simulink model "sm_trackV_belt4_IdlerArm_i2u0r3"  (R2026b)
settings: Solver=ode23t  StopTime=14  AbsTol=1e-3  EnableMultiTasking=on
PostLoadFcn:
  | sm_trackV_measure_loads([bdroot '/Track FL'],'Actuator Torque')
  | sm_trackV_measure_loads([bdroot '/Track FR'],'Actuator Torque')
  | sm_trackV_measure_loads([bdroot '/Track RL'],'Actuator Torque')
  | sm_trackV_measure_loads([bdroot '/Track RR'],'Actuator Torque')
StartFcn:
  | tic
StopFcn:
  | Elapsed_Sim_Time = toc;
  | disp(['Elapsed Sim Time = ' num2str(Elapsed_Sim_Time)]);
undefined symbols (not defined in the file): X, Y, Z
libraries: sm_lib x9, fl_lib x8, nesl_utility x5, sm_trackV_lib_chain_underc_elem x4, simulink x4, sm_trackV_lib_belt_lower_frame_s45i2u0l3 x4, sm_excv_chassis_lib x3, sm_trackV_lib_terrain_contact x3
settings Model: Creator=smiller  LastModifiedBy=smiller
settings SolverCC: AutoScaleAbsTol=off
settings DataIOCC: LimitDataPoints=on  MaxDataPoints=10000  ReturnWorkspaceOutputs=off  SignalLoggingName=logsout_sm_trackV_belt4_IdlerArm_i2u0r3
settings OptimizationCC: LifeSpan=inf  ReuseModelBlockBuffer=off
settings DebuggingCC: AllowSymbolicDim=off  ArithmeticOperatorsInVariantConditions=warning  SFExecutionAtInitializationDiag=none  SFNoUnconditionalDefaultTransitionDiag=warning  SFUnexpectedBacktrackingDiag=warning  SubsystemReferenceDiagnosticForUnitTest=warning
settings SFSimCC: CustomCodeUndefinedFunction=UseInterfaceOnly  SimUseLocalCustomCode=off
settings RTWCC: DLArmComputeVersion=19.05  RTWUseLocalCustomCode=off
settings CodeAppCC: StateflowObjectComments=on
settings GRTTargetCC: TargetLangStandard=C89/C90 (ANSI)
settings ConfigComp: CovExternalEMLEnable=off  CovSFcnEnable=off  CovSaveCumulativeToWorkspaceVar=on  CovSaveSingleToWorkspaceVar=on
settings SimscapeCC: SimscapeLogLimitData=off  SimscapeLogName=simlog_sm_trackV_belt4_IdlerArm_i2u0r3  SimscapeLogSimulationStatistics=on  SimscapeLogType=all  SimscapeUseEnergyAccounting=off
settings DiagnosticsConfigSet: SimMechanicsConflictingReferenceFrames=none  SimMechanicsUnconnectedFramePorts=none
settings ExplorerConfigSet: InternalSimMechanicsExplorerSettings="<ExplorerConfiguration><canonicalview>default</canonicalview><AnimationSetting><BasePlaybackSpeed>1.0</BasePlaybackSpeed><PlaybackSpeedFactor>4.0</PlaybackSpeedFactor></AnimationSetting><TilePanel><TileInfo><Tiles Columns=\"2\" Count=\"3\" Rows=\"2\"><Column Weight=\"0.5\"/><Column Weight=\"0.5\"/><Row Weight=\"0.4992\"/><Row Weight=\"0.5008\"/><Tile Height=\"2\" Width=\"1\" X=\"0\" Y=\"0\"/><Tile Height=\"1\" Width=\"1\" X=\"1\" Y=\"0\"/><Tile Height=\"1\" Width=\"1\" X=\"1\" Y=\"1\"/></Tiles></TileInfo><SceneInfo><SceneViewer><BGColor><R>1</R><G>1</G><B>1</B></BGColor><Camera><DoPerspective>on</DoPerspective><Position><X>8</X><Y>-4.69999999999999929</Y><Z>3.49999999999999956</Z></Position><Center><X>7.32379042217759135</X><Y>-4.02379042217759064</Y><Z>3.20762829527726279</Z></Center><Up><X>0</X><Y>0</Y><Z>1</Z></Up><ViewLimDist>1</ViewLimDist><YLim>0.466307658154998583</YLim><XLim>0.48985854998100864</XLim></Camera></SceneViewer><SceneViewer><BGColor><R>1</R><G>1</G><B>1</B></BGColor><Camera><DoPerspective>on</DoPerspective><Position><X>0</X><Y>-3.99999999999999911</Y><Z>1.09999999999999964</Z></Position><Center><X>2.22044604925031308e-16</X><Y>-2.99999999999999911</Y><Z>1.09999999999999964</Z></Center><Up><X>0</X><Y>0</Y><Z>1</Z></Up><ViewLimDist>1</ViewLimDist><YLim>0.466307658154998583</YLim><XLim>0.996493077701092966</XLim></Camera></SceneViewer><SceneViewer><BGColor><R>1</R><G>1</G><B>1</B></BGColor><Camera><DoPerspective>on</DoPerspective><Position><X>2</X><Y>8.88178419700125232e-16</Y><Z>9</Z></Position><Center><X>2</X><Y>8.88178419700125232e-16</Y><Z>8</Z></Center><Up><X>0</X><Y>1</Y><Z>0</Z></Up><ViewLimDist>1</ViewLimDist><YLim>0.466307658154998583</YLim><XLim>0.993092077435901444</XLim></Camera></SceneViewer></SceneInfo></TilePanel><MechEditorPanel><Cameras><Camera><Id>Camera1</Id><Value><Name>Track_CtrRear_AimFront</Name><NativeCamera><PositionTrackingFeature>Chassis.Camera_Frames.CamF_CtrRear_AimLF.R</PositionTrackingFeature><CenterTrackingFeature>Config.World_Frame.W</CenterTrackingFeature><UpVectorTrackingFeature>Config.World_Frame.W</UpVectorTrackingFeature><CenterTrackingOrigin>off</CenterTrackingOrigin><CenterTrackingDirection>+X</CenterTrackingDirection><UpVectorTrackingDirection>+Z</UpVectorTrackingDirection></NativeCamera></Value></Camera><Camera><Id>Camera2</Id><Value><Name>Track_Left_AimRight</Name><NativeCamera><PositionTrackingFeature>Chassis.Camera_Frames.CamF_Left_AimRight.R</PositionTrackingFeature><CenterTrackingFeature>Chassis.Camera_Frames.CamF_Left_AimRight.R</CenterTrackingFeature><UpVectorTrackingFeature>Config.World_Frame.W</UpVectorTrackingFeature><CenterTrackingOrigin>off</CenterTrackingOrigin><CenterTrackingDirection>+X</CenterTrackingDirection><UpVectorTrackingDirection>+Z</UpVectorTrackingDirection></NativeCamera></Value></Camera><Camera><Id>Camera3</Id><Value><Name>Track_Front_AimLR</Name><NativeCamera><PositionTrackingFeature>Chassis.Camera_Frames.CamF_Front_AimLR.R</PositionTrackingFeature><CenterTrackingFeature>Chassis.Camera_Frames.Transform_Front_AimLR.F</CenterTrackingFeature><UpVectorTrackingFeature>Config.World_Frame.W</UpVectorTrackingFeature><CenterTrackingOrigin>off</CenterTrackingOrigin><CenterTrackingDirection>+X</CenterTrackingDirection><UpVectorTrackingDirection>+Z</UpVectorTrackingDirection></NativeCamera></Value></Camera><Camera><Id>Camera4</Id><Value><Name>Track_Right_AimLeftTL</Name><NativeCamera><PositionTrackingFeature>Chassis.Camera_Frames.CamF_Right_AimLeftTL.R</PositionTrackingFeature><CenterTrackingFeature>Chassis.Camera_Frames.CamF_Right_AimLeftTL.R</CenterTrackingFeature><UpVectorTrackingFeature>Config.World_Frame.W</UpVectorTrackingFeature><CenterTrackingOrigin>off</CenterTrackingOrigin><CenterTrackingDirection>+X</CenterTrackingDirection><UpVectorTrackingDirection>+Z</UpVectorTrackingDirection></NativeCamera></Value></Camera><Camera><Id>Camera5</Id><Value><Name>Track_Right_AimLeftTR</Name><NativeCamera><PositionTrackingFeature>Chassis.Camera_Frames.CamF_Right_AimLeftTR.R</PositionTrackingFeature><CenterTrackingFeature>Chassis.Camera_Frames.CamF_Right_AimLeftTR.R</CenterTrackingFeature><UpVectorTrackingFeature>Config.World_Frame.W</UpVectorTrackingFeature><CenterTrackingOrigin>off</CenterTrackingOrigin><CenterTrackingDirection>+X</CenterTrackingDirection><UpVectorTrackingDirection>+Z</UpVectorTrackingDirection></NativeCamera></Value></Camera><Camera><Id>Camera6</Id><Value><Name>Track_FR_AimFront</Name><NativeCamera><PositionTrackingFeature>Chassis.Camera_Frames.CamF_FR_Aim_Front_R</PositionTrackingFeature><CenterTrackingFeature>Chassis.Camera_Frames.CamF_FR_Aim_Front_R</CenterTrackingFeature><UpVectorTrackingFeature>Config.W</UpVectorTrackingFeature><CenterTrackingOrigin>off</CenterTrackingOrigin><CenterTrackingDirection>+X</CenterTrackingDirection><UpVectorTrackingDirection>+Z</UpVectorTrackingDirection></NativeCamera></Value></Camera><Camera><Id>Camera7</Id><Value><Name>TrackIsoFR</Name><NativeCamera><PositionKeyframeSet><Keyframe><Time>0</Time><Value><X>7.6744465174951229</X><Y>-7.3378434494995588</Y><Z>0.83192924808838675</Z></Value></Keyframe><Keyframe><Time>4.8580359639439301</Time><Value><X>7.6744465174951229</X><Y>-7.3378434494995588</Y><Z>0.83192924808838675</Z></Value></Keyframe><Keyframe><Time>7.0422197385672698</Time><Value><X>8.4041500304882533</X><Y>-6.0478565656515233</Y><Z>1.2378387423585568</Z></Value></Keyframe><Keyframe><Time>12.78196840006439</Time><Value><X>20.29732183415512</X><Y>-9.1045432763174095</Y><Z>1.6217023498793322</Z></Value></Keyframe></PositionKeyframeSet><CenterKeyframeSet><Keyframe><Time>0</Time><Value><X>-3.9707986865367024</X><Y>13.1242688081241</Y><Z>1.8580696339996621</Z></Value></Keyframe><Keyframe><Time>4.8580359639439301</Time><Value><X>4.507312599752261</X><Y>-1.7728039312810333</Y><Z>1.1110065851169071</Z></Value></Keyframe><Keyframe><Time>7.0422197385672698</Time><Value><X>6.9754199629584264</X><Y>-2.3648388994835718</Y><Z>1.2924635728623486</Z></Value></Keyframe><Keyframe><Time>12.78196840006439</Time><Value><X>16.536524754348189</X><Y>-2.4963653739311518</Y><Z>1.9530913158644347</Z></Value></Keyframe></CenterKeyframeSet><UpVectorKeyframeSet><Keyframe><Time>0</Time><Value><X>0.036204453435340365</X><Y>-0.029489201528742272</Y><Z>0.99890921736894867</Z></Value></Keyframe><Keyframe><Time>4.8580359639439301</Time><Value><X>0.036204453435340372</X><Y>-0.029489201528742279</Y><Z>0.99890921736894867</Z></Value></Keyframe><Keyframe><Time>7.0422197385672698</Time><Value><X>0.015774113925201387</X><Y>-0.0087099802030477149</Y><Z>0.99983764360756966</Z></Value></Keyframe><Keyframe><Time>12.78196840006439</Time><Value><X>0.036204453435340372</X><Y>-0.029489201528742286</Y><Z>0.99890921736894867</Z></Value></Keyframe></UpVectorKeyframeSet></NativeCamera></Value></Camera><Camera><Id>Camera8</Id><Value><Name>Track_IsoFR_Big</Name><NativeCamera><PositionTrackingFeature>Chassis.Camera_Frames.CamF_FR_AimCtr_Big.R</PositionTrackingFeature><CenterTrackingFeature>Chassis.Camera_Frames.CamF_FR_AimCtr_Big.R</CenterTrackingFeature><UpVectorTrackingFeature>Config.W.frame</UpVectorTrackingFeature><CenterTrackingOrigin>off</CenterTrackingOrigin><CenterTrackingDirection>+X</CenterTrackingDirection><UpVectorTrackingDirection>+Z</UpVectorTrackingDirection></NativeCamera></Value></Camera><Camera><Id>Camera9</Id><Value><Name>Track_Top_FixO</Name><NativeCamera><PositionTrackingFeature>Chassis.Camera_Frames.CamF_Top.R</PositionTrackingFeature><CenterTrackingFeature>Config.W</CenterTrackingFeature><UpVectorTrackingFeature>Config.W</UpVectorTrackingFeature><CenterTrackingOrigin>off</CenterTrackingOrigin><CenterTrackingDirection>-Z</CenterTrackingDirection><UpVectorTrackingDirection>+Y</UpVectorTrackingDirection></NativeCamera></Value></Camera><Camera><Id>Camera10</Id><Value><Name>Track_Terrain_Steer</Name><NativeCamera><PositionKeyframeSet><Keyframe><Time>1.954306185234983</Time><Value><X>6.8114446186923496</X><Y>-5.3171553607278206</Y><Z>2.3434891046120194</Z></Value></Keyframe><Keyframe><Time>3.2620190833091063</Time><Value><X>8.6993949048857981</X><Y>-5.3317331728841273</Y><Z>2.4343360662333233</Z></Value></Keyframe><Keyframe><Time>5.0400013056141875</Time><Value><X>10.892348868797249</X><Y>-5.3777629823446311</Y><Z>2.9548739629979583</Z></Value></Keyframe><Keyframe><Time>6.4399956757078574</Time><Value><X>12.590773161836934</X><Y>-5.02192612890686</Y><Z>3.4550574594673802</Z></Value></Keyframe><Keyframe><Time>8.274080048576554</Time><Value><X>14.467163111987707</X><Y>-3.5325878594240057</Y><Z>3.6687375492730663</Z></Value></Keyframe><Keyframe><Time>10.611771973115053</Time><Value><X>16.092056497155664</X><Y>-0.19034994331009364</Y><Z>3.5642210119966649</Z></Value></Keyframe><Keyframe><Time>12.781922870204893</Time><Value><X>16.438502065245114</X><Y>2.6045222313399137</Y><Z>3.7512090554216835</Z></Value></Keyframe><Keyframe><Time>14</Time><Value><X>15.821419267246833</X><Y>4.405488260701441</Y><Z>3.6561806172412985</Z></Value></Keyframe></PositionKeyframeSet><CenterKeyframeSet><Keyframe><Time>1.954306185234983</Time><Value><X>3.8269446610796178</X><Y>-1.4237791566024609</Y><Z>1.4146779468278596</Z></Value></Keyframe><Keyframe><Time>3.2620190833091063</Time><Value><X>5.6599243323637811</X><Y>-1.3666460332407318</Y><Z>1.4884174126531708</Z></Value></Keyframe><Keyframe><Time>5.0400013056141875</Time><Value><X>7.9655341663497534</X><Y>-1.5596390492794066</Y><Z>2.0440151286844124</Z></Value></Keyframe><Keyframe><Time>6.4399956757078574</Time><Value><X>8.8172775775206471</X><Y>-0.099279748271351664</Y><Z>2.280701670444107</Z></Value></Keyframe><Keyframe><Time>8.274080048576554</Time><Value><X>11.140862936281749</X><Y>0.80667772469433485</Y><Z>2.633554181468174</Z></Value></Keyframe><Keyframe><Time>10.611771973115053</Time><Value><X>12.246653975093967</X><Y>4.8261013508136488</Y><Z>2.3674869461938366</Z></Value></Keyframe><Keyframe><Time>12.781922870204893</Time><Value><X>13.419912109075547</X><Y>6.5423699352357101</Y><Z>2.8117886929204419</Z></Value></Keyframe><Keyframe><Time>14</Time><Value><X>13.045484539267546</X><Y>8.0267844133623925</Y><Z>2.7922773888123493</Z></Value></Keyframe></CenterKeyframeSet><UpVectorKeyframeSet><Keyframe><Time>1.954306185234983</Time><Value><X>-0.1264530356370476</X><Y>0.13743109156705063</Y><Z>0.98240639495519599</Z></Value></Keyframe><Keyframe><Time>3.2620190833091063</Time><Value><X>-0.1264530356370476</X><Y>0.13743109156705063</Y><Z>0.98240639495519599</Z></Value></Keyframe><Keyframe><Time>5.0400013056141875</Time><Value><X>-0.12645303563704768</X><Y>0.13743109156705072</Y><Z>0.98240639495519599</Z></Value></Keyframe><Keyframe><Time>6.4399956757078574</Time><Value><X>-0.12645303563704768</X><Y>0.13743109156705072</Y><Z>0.98240639495519599</Z></Value></Keyframe><Keyframe><Time>8.274080048576554</Time><Value><X>-0.12645303563704768</X><Y>0.13743109156705069</Y><Z>0.98240639495519611</Z></Value></Keyframe><Keyframe><Time>10.611771973115053</Time><Value><X>-0.12645303563704768</X><Y>0.13743109156705069</Y><Z>0.98240639495519599</Z></Value></Keyframe><Keyframe><Time>12.781922870204893</Time><Value><X>-0.12645303563704771</X><Y>0.13743109156705072</Y><Z>0.98240639495519599</Z></Value></Keyframe><Keyframe><Time>14</Time><Value><X>-0.12645303563704774</X><Y>0.13743109156705072</Y><Z>0.98240639495519588</Z></Value></Keyframe></UpVectorKeyframeSet></NativeCamera></Value></Camera></Cameras><GfxPanelCameraMap><MapElement CameraMLId=\"Camera8\" GfxPanelIndex=\"0\"/><MapElement CameraMLId=\"Camera5\" GfxPanelIndex=\"1\"/><MapElement CameraMLId=\"Camera9\" GfxPanelIndex=\"2\"/></GfxPanelCameraMap><VideoCreator><PlaybackSpeedRatio>0.5</PlaybackSpeedRatio><FrameRate>30</FrameRate><VideoFormat>MPEG-4</VideoFormat><FrameSize>auto</FrameSize></VideoCreator></MechEditorPanel></ExplorerConfiguration>"

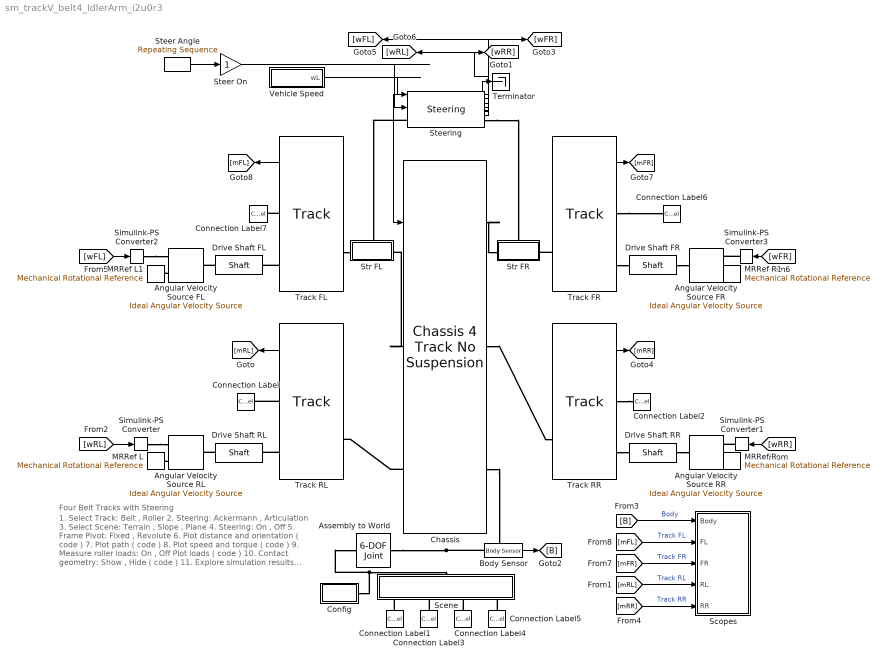
== system sm_trackV_belt4_IdlerArm_i2u0r3 ==
  note: 1. Select Track: Belt , Roller
      | 2. Steering: Ackermann , Articulation
      | 3. Select Scene: Terrain , Slope , Plane
      | 4. Steering: On , Off
      | 5. Frame Pivot: Fixed , Revolute
      | 6. Plot distance and orientation ( code )
      | 7. Plot path ( code )
      | 8. Plot speed and torque ( code )
      | 9. Measure roller loads: On , Off Plot loads ( code )
      | 10. Contact geometry: Show , Hide ( code )
      | 11. Explore simulation results using sscexplore
      | 12. Learn more about this example
  note: Four Belt Tracks with Steering
  Angular Velocity Source FL : fl_lib/Mechanical/Mechanical Sources/Ideal Angular Velocity Source
  Angular Velocity Source FR : fl_lib/Mechanical/Mechanical Sources/Ideal Angular Velocity Source
  Angular Velocity Source RL : fl_lib/Mechanical/Mechanical Sources/Ideal Angular Velocity Source
  Angular Velocity Source RR : fl_lib/Mechanical/Mechanical Sources/Ideal Angular Velocity Source
  Assembly to World : sm_lib/Joints/6-DOF Joint  JointMode=Normal  CompositeWrenchDir=FollowerOnBase  CompositeWrenchFrame=BaseFrame  SenseConstraintForce=off  SenseConstraintTorque=off  SenseTotalForce=off  SenseTotalTorque=off  PxPositionTargetSpecify=on  PxPositionTargetPriority=High  PxPositionTargetValue=0  PxPositionTargetValueUnits=m  PxVelocityTargetSpecify=off  PxVelocityTargetPriority=High  PxVelocityTargetValue=0  PxVelocityTargetValueUnits=m/s  PxEquilibriumPosition=0  PxEquilibriumPositionUnits=m  PxSpringStiffness=0  PxSpringStiffnessUnits=N/m  PxDampingCoefficient=0  PxDampingCoefficientUnits=N/(m/s)  PxLowerLimitSpecify=off  PxLowerLimitBound=-1  PxLowerLimitBoundUnits=m  PxLowerLimitStiffness=1e6  PxLowerLimitStiffnessUnits=N/m  PxLowerLimitDamping=1e3  PxLowerLimitDampingUnits=N/(m/s)  PxLowerLimitTransitionRegionWidth=1e-4  PxLowerLimitTransitionRegionWidthUnits=m  PxUpperLimitSpecify=off  PxUpperLimitBound=1  PxUpperLimitBoundUnits=m  PxUpperLimitStiffness=1e6  PxUpperLimitStiffnessUnits=N/m  PxUpperLimitDamping=1e3  PxUpperLimitDampingUnits=N/(m/s)  PxUpperLimitTransitionRegionWidth=1e-4  PxUpperLimitTransitionRegionWidthUnits=m  PxTorqueActuationMode=NoTorque  PxMotionActuationMode=ComputedMotion  PxSensePosition=off  PxSenseVelocity=off  PxSenseAcceleration=off  PxSenseTorqueForce=off  PxSenseLowerLimitTorqueForce=off  PxSenseUpperLimitTorqueForce=off  PyPositionTargetSpecify=on  PyPositionTargetPriority=High  PyPositionTargetValue=0  PyPositionTargetValueUnits=m  PyVelocityTargetSpecify=off  PyVelocityTargetPriority=High  PyVelocityTargetValue=0  PyVelocityTargetValueUnits=m/s  PyEquilibriumPosition=0  PyEquilibriumPositionUnits=m  PySpringStiffness=0  PySpringStiffnessUnits=N/m  PyDampingCoefficient=0  PyDampingCoefficientUnits=N/(m/s)  PyLowerLimitSpecify=off  PyLowerLimitBound=-1  PyLowerLimitBoundUnits=m  PyLowerLimitStiffness=1e6  PyLowerLimitStiffnessUnits=N/m  PyLowerLimitDamping=1e3  PyLowerLimitDampingUnits=N/(m/s)  PyLowerLimitTransitionRegionWidth=1e-4  PyLowerLimitTransitionRegionWidthUnits=m  PyUpperLimitSpecify=off  PyUpperLimitBound=1  PyUpperLimitBoundUnits=m  PyUpperLimitStiffness=1e6  PyUpperLimitStiffnessUnits=N/m  PyUpperLimitDamping=1e3  PyUpperLimitDampingUnits=N/(m/s)  PyUpperLimitTransitionRegionWidth=1e-4  PyUpperLimitTransitionRegionWidthUnits=m  PyTorqueActuationMode=NoTorque  PyMotionActuationMode=ComputedMotion  PySensePosition=off  PySenseVelocity=off  PySenseAcceleration=off  PySenseTorqueForce=off  PySenseLowerLimitTorqueForce=off  PySenseUpperLimitTorqueForce=off  PzPositionTargetSpecify=on  PzPositionTargetPriority=High  PzPositionTargetValue=1.5  PzPositionTargetValueUnits=m  PzVelocityTargetSpecify=off  PzVelocityTargetPriority=High  PzVelocityTargetValue=0  PzVelocityTargetValueUnits=m/s  PzEquilibriumPosition=0  PzEquilibriumPositionUnits=m  PzSpringStiffness=0  PzSpringStiffnessUnits=N/m  PzDampingCoefficient=0  PzDampingCoefficientUnits=N/(m/s)  PzLowerLimitSpecify=off  PzLowerLimitBound=-1  PzLowerLimitBoundUnits=m  PzLowerLimitStiffness=1e6  PzLowerLimitStiffnessUnits=N/m  PzLowerLimitDamping=1e3  PzLowerLimitDampingUnits=N/(m/s)  PzLowerLimitTransitionRegionWidth=1e-4  PzLowerLimitTransitionRegionWidthUnits=m  PzUpperLimitSpecify=off  PzUpperLimitBound=1  PzUpperLimitBoundUnits=m  PzUpperLimitStiffness=1e6  PzUpperLimitStiffnessUnits=N/m  PzUpperLimitDamping=1e3  PzUpperLimitDampingUnits=N/(m/s)  PzUpperLimitTransitionRegionWidth=1e-4  PzUpperLimitTransitionRegionWidthUnits=m  PzTorqueActuationMode=NoTorque  PzMotionActuationMode=ComputedMotion  PzSensePosition=off  PzSenseVelocity=off  PzSenseAcceleration=off  PzSenseTorqueForce=off  PzSenseLowerLimitTorqueForce=off  PzSenseUpperLimitTorqueForce=off  SphPositionTargetSpecify=off  SphPositionTargetPriority=High  SphPositionTargetRotationMethod=StandardAxis  SphPositionTargetFollAlignAxisA=+X  SphPositionTargetBaseAlignAxisA=+Y  SphPositionTargetFollAlignAxisB=+Y  SphPositionTargetBaseAlignAxisB=+Z  SphPositionTargetRotationStandardAxis=+Z  SphPositionTargetRotationAngle=180  SphPositionTargetRotationAngleUnits=deg  SphPositionTargetRotationArbitraryAxis=[0 0 1]  SphPositionTargetRotationSequenceAxes=FollowerAxes  SphPositionTargetRotationSequence=XYX  SphPositionTargetRotationSequenceAngles=[0 0 0]  SphPositionTargetRotationSequenceAnglesUnits=deg  SphPositionTargetRotationMatrix=[1 0 0; 0 1 0; 0 0 1]  SphPositionTargetQuaternion=[1 0 0 0]  SphVelocityTargetSpecify=off  SphVelocityTargetPriority=High  SphVelocityTargetValue=[0 0 0]  SphVelocityTargetValueUnits=deg/s  SphVelocityTargetInFollowerFrame=on  SphEqPosRotationMethod=None  SphEqPosFollAlignAxisA=+X  SphEqPosBaseAlignAxisA=+Y  SphEqPosFollAlignAxisB=+Y  SphEqPosBaseAlignAxisB=+Z  SphEqPosRotationStandardAxis=+Z  SphEqPosRotationAngle=0.0  SphEqPosRotationAngleUnits=deg  SphEqPosRotationArbitraryAxis=[0 0 1]  SphEqPosRotationSequenceAxes=FollowerAxes  SphEqPosRotationSequence=XYX  SphEqPosRotationSequenceAngles=[0 0 0]  SphEqPosRotationSequenceAnglesUnits=deg  SphEqPosRotationMatrix=[1 0 0; 0 1 0; 0 0 1]  SphEqPosQuaternion=[1 0 0 0]  SphSpringStiffness=0  SphSpringStiffnessUnits=N*m/deg  SphDampingCoefficient=0  SphDampingCoefficientUnits=N*m/(deg/s)  SphLowerLimitSpecify=off  SphLowerLimitBound=15  SphLowerLimitBoundUnits=deg  SphLowerLimitStiffness=1e4  SphLowerLimitStiffnessUnits=N*m/deg  SphLowerLimitDamping=10  SphLowerLimitDampingUnits=N*m/(deg/s)  SphLowerLimitTransitionRegionWidth=0.1  SphLowerLimitTransitionRegionWidthUnits=deg  SphUpperLimitSpecify=off  SphUpperLimitBound=45  SphUpperLimitBoundUnits=deg  SphUpperLimitStiffness=1e4  SphUpperLimitStiffnessUnits=N*m/deg  SphUpperLimitDamping=10  SphUpperLimitDampingUnits=N*m/(deg/s)  SphUpperLimitTransitionRegionWidth=0.1  SphUpperLimitTransitionRegionWidthUnits=deg  SphTorqueActuationMode=NoTorque  SphActuateTorqueX=off  SphActuateTorqueY=off  SphActuateTorqueZ=off  SphActuateTorque=off  SphActuationFrame=BaseFrame  SphSensePosition=off  SphSenseVelocityX=off  SphSenseVelocityY=off  SphSenseVelocityZ=off  SphSenseVelocity=off  SphSenseAccelerationX=off  SphSenseAccelerationY=off  SphSenseAccelerationZ=off  SphSenseAcceleration=off  SphSenseLowerLimitTorqueMag=off  SphSenseUpperLimitTorqueMag=off  SphSensingFrame=BaseFrame
  Body Sensor : sm_excv_chassis_lib/Body Sensor  offset_body_sensor=[0 0 0]
  Chassis : sm_excv_chassis_lib/Chassis 4 Track No Suspension  popup_chassis_geo=CAD Shell
  Config : Subsystem
  Connection Label : ConnectionLabel  Label=GFL
  Connection Label1 : ConnectionLabel  Label=GFL
  Connection Label2 : ConnectionLabel  Label=GFR
  Connection Label3 : ConnectionLabel  Label=GFR
  Connection Label4 : ConnectionLabel  Label=GRL
  Connection Label5 : ConnectionLabel  Label=GRR
  Connection Label6 : ConnectionLabel  Label=GRR
  Connection Label7 : ConnectionLabel  Label=GRL
  Drive Shaft FL : sm_trackV_lib_chain_underc_elem/Shaft  k_shaft=Excv.Drive.Shaft.k  b_shaft=Excv.Drive.Shaft.b
  Drive Shaft FR : sm_trackV_lib_chain_underc_elem/Shaft  k_shaft=Excv.Drive.Shaft.k  b_shaft=Excv.Drive.Shaft.b
  Drive Shaft RL : sm_trackV_lib_chain_underc_elem/Shaft  k_shaft=Excv.Drive.Shaft.k  b_shaft=Excv.Drive.Shaft.b
  Drive Shaft RR : sm_trackV_lib_chain_underc_elem/Shaft  k_shaft=Excv.Drive.Shaft.k  b_shaft=Excv.Drive.Shaft.b
  MRRef L : fl_lib/Mechanical/Rotational Elements/Mechanical Rotational Reference
  MRRef L1 : fl_lib/Mechanical/Rotational Elements/Mechanical Rotational Reference
  MRRef R : fl_lib/Mechanical/Rotational Elements/Mechanical Rotational Reference
  MRRef R1 : fl_lib/Mechanical/Rotational Elements/Mechanical Rotational Reference
  Scene : Subsystem  Variant=on  VariantControlMode=label  VariantControl=Terrain  LabelModeActiveChoice=Terrain
      settings: AttributesFormatString=%<LabelModeActiveChoice>
      mask Display: disp(' ')
  Scopes : Subsystem
  Simulink-PS Converter{,1..3} (4 alike) : nesl_utility/Simulink-PS Converter  PhysicalDomain=network_engine_domain  SubClassName=ps_input  LeftPortType=input  RightPortType=output  PseudoPeriodic=off  Frequencies=[]  NoiseDistribution=none  NoiseParameters=[]  Unit=1  AffineConversion=off  FilteringAndDerivatives=provide  SimscapeFilterOrder=1  InputFilterTimeConstant=0.001  UdotUserProvided=0
  Steer Angle : simulink/Sources/Repeating Sequence  rep_seq_t="[0 3  5  14 16 18  20  29 31 36]"  rep_seq_y="[0 0 20 20  0   0 -20 -20  0   0]*pi/180"
  Steer On : Gain
  Steering : sm_excv_chassis_lib/Steering  popup_steering=Ackermann  yTrack=Trac.Chassis.Front.TrackSepCtr  steerRatio=1  tcSteer=0.1  wheelbase=Trac.Chassis.AxleSeparation
      settings: AttributesFormatString=%<popup_steering>
  Str FL : Subsystem
      settings: PortSchema="{\"entries\":[{\"content\":{\"sides\":[{\"content\":{\"connectorIds\":[\"LConn1\"]},\"type\":\"ConnectorPlacement.EquallySpacedRectSide\",\"uuid\":\"c7c7e178-8ee1-427d-9e3f-0887a6c2686c\"},{\"content\":{\"connectorIds\":[\"RConn1\"],\"side\":\"RIGHT\"},\"type\":\"ConnectorPlacement.EquallySpacedRectSide\",\"uuid\":\"0bc250c9-893f-4ff8-8fb1-de52c2b7a8cd\"},{\"content\":{\"connectorIds\":[\"LConn2\"],\"side\":\"TOP\"},\"type\":\"ConnectorPlacement.EquallySpacedRectSide\",\"uuid\":\"31ffd3a3-da84-490a-ac6f-43ff5d5145cd\"}]},\"type\":\"ConnectorPlacement.EquallySpacedConnector\",\"uuid\":\"2f775820-965f-444f-9db7-4d7e95d78bbe\"}],\"packageUris\":[\"http://schema.mathworks.com/mf0/Connector/R2020b\"],\"version\":\"1.0\"}"
  Str FR : Subsystem
      settings: PortSchema="{\"entries\":[{\"content\":{\"sides\":[{\"content\":{\"connectorIds\":[\"LConn1\"]},\"type\":\"ConnectorPlacement.EquallySpacedRectSide\",\"uuid\":\"c7c7e178-8ee1-427d-9e3f-0887a6c2686c\"},{\"content\":{\"connectorIds\":[\"RConn1\"],\"side\":\"RIGHT\"},\"type\":\"ConnectorPlacement.EquallySpacedRectSide\",\"uuid\":\"0bc250c9-893f-4ff8-8fb1-de52c2b7a8cd\"},{\"content\":{\"connectorIds\":[\"LConn2\"],\"side\":\"TOP\"},\"type\":\"ConnectorPlacement.EquallySpacedRectSide\",\"uuid\":\"31ffd3a3-da84-490a-ac6f-43ff5d5145cd\"}]},\"type\":\"ConnectorPlacement.EquallySpacedConnector\",\"uuid\":\"2f775820-965f-444f-9db7-4d7e95d78bbe\"}],\"packageUris\":[\"http://schema.mathworks.com/mf0/Connector/R2020b\"],\"version\":\"1.0\"}"
  Terminator : Terminator
  Track FL : sm_trackV_lib_belt_lower_frame_s45i2u0l3/Track  LabelModeActiveChoice=BeltPts  popup_trackModel=Belt, Points  popup_leftOrRight=Left  popup_sense_roller=Actuator Torque  popup_trackFrame=Fixed
      settings: AttributesFormatString=%<popup_trackFrame>, %<popup_sense_roller>
  Track FR : sm_trackV_lib_belt_lower_frame_s45i2u0l3/Track  LabelModeActiveChoice=BeltPts  popup_trackModel=Belt, Points  popup_leftOrRight=Right  popup_sense_roller=Actuator Torque  popup_trackFrame=Fixed
      settings: AttributesFormatString=%<popup_trackFrame>, %<popup_sense_roller>
  Track RL : sm_trackV_lib_belt_lower_frame_s45i2u0l3/Track  LabelModeActiveChoice=BeltPts  popup_trackModel=Belt, Points  popup_leftOrRight=Left  popup_sense_roller=Actuator Torque  popup_trackFrame=Fixed
      settings: AttributesFormatString=%<popup_trackFrame>, %<popup_sense_roller>
  Track RR : sm_trackV_lib_belt_lower_frame_s45i2u0l3/Track  LabelModeActiveChoice=BeltPts  popup_trackModel=Belt, Points  popup_leftOrRight=Right  popup_sense_roller=Actuator Torque  popup_trackFrame=Fixed
      settings: AttributesFormatString=%<popup_trackFrame>, %<popup_sense_roller>
  Vehicle Speed : Subsystem  Variant=on  VariantControlMode=label  VariantControl=Choice  LabelModeActiveChoice=Fwd
      settings: AttributesFormatString=%<LabelModeActiveChoice>
      mask Display: disp(' ')
  wires:
  Track RL/1 -> [mRL]
  Body Sensor/1 -> [B]
  Vehicle Speed/1(wL) -> Steering/1
  [B] -> Scopes/1(Body)  "Body"
  [mRR] -> Scopes/5(RR)  "Track RR"
  [mRL] -> Scopes/4(RL)  "Track RL"
  Track RR/1 -> [mRR]
  Steer Angle/1 -> Steer On/1
  Steering/4 -> [wFR]
  Steering/3 -> [wFL]
  [wFR] -> Simulink-PS Converter3/1
  [wFL] -> Simulink-PS Converter2/1
  Steering/2 -> [wRL]
  Steering/5 -> [wRR]
  [wRR] -> Simulink-PS Converter1/1
  [wRL] -> Simulink-PS Converter/1
  Steering/6 -> Terminator/1
  Track FR/1 -> [mFR]
  Track FL/1 -> [mFL]
  [mFL] -> Scopes/2(FL)  "Track FL"
  [mFR] -> Scopes/3(FR)  "Track FR"
  Steer On/1 -> Steering/2
  Steering/1 -> Chassis/1
  connections:
  Chassis/RConn2 -- Track RR/LConn2
  Chassis/LConn2 -- Track RL/LConn2
  Track RL/RConn1 -- Connection Label/LConn1
  Track RR/RConn1 -- Connection Label2/LConn1
  Simulink-PS Converter1/RConn1 -- Angular Velocity Source RR/RConn1
  Angular Velocity Source RR/RConn2 -- MRRef R/LConn1
  Track RL/RConn2 -- Drive Shaft RL/RConn1
  Drive Shaft RR/LConn1 -- Angular Velocity Source RR/LConn1
  Track RR/RConn2 -- Drive Shaft RR/RConn1
  Simulink-PS Converter/RConn1 -- Angular Velocity Source RL/RConn1
  Angular Velocity Source RL/RConn2 -- MRRef L/LConn1
  Drive Shaft RL/LConn1 -- Angular Velocity Source RL/LConn1
  Config/LConn1 -- Assembly to World/LConn1 -- Scene/RConn1
  Chassis/LConn1 -- Str FL/LConn1
  Angular Velocity Source FL/RConn2 -- MRRef L1/LConn1
  Simulink-PS Converter2/RConn1 -- Angular Velocity Source FL/RConn1
  Track FL/RConn2 -- Drive Shaft FL/RConn1
  Drive Shaft FL/LConn1 -- Angular Velocity Source FL/LConn1
  Track FR/RConn2 -- Drive Shaft FR/RConn1
  Drive Shaft FR/LConn1 -- Angular Velocity Source FR/LConn1
  Angular Velocity Source FR/RConn2 -- MRRef R1/LConn1
  Simulink-PS Converter3/RConn1 -- Angular Velocity Source FR/RConn1
  Track FR/RConn1 -- Connection Label6/LConn1
  Track FL/RConn1 -- Connection Label7/LConn1
  Chassis/RConn1 -- Str FR/LConn1
  Track FR/LConn2 -- Str FR/RConn1
  Track FL/LConn2 -- Str FL/RConn1
  Steering/LConn1 -- Str FL/LConn2
  Steering/RConn1 -- Str FR/LConn2
  Assembly to World/RConn1 -- Chassis/RConn3 -- Body Sensor/LConn1
  Connection Label1/LConn1 -- Scene/LConn1
  Connection Label3/LConn1 -- Scene/LConn2
  Connection Label4/LConn1 -- Scene/LConn3
  Connection Label5/LConn1 -- Scene/LConn4

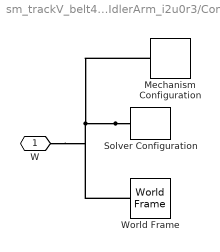
== system sm_trackV_belt4_IdlerArm_i2u0r3/Config ==
  Mechanism Configuration : sm_lib/Utilities/Mechanism Configuration  UniformGravity=Constant  GravityVector=[0 0 -9.80665]  GravityVectorUnits=m/s^2  LinearizationDelta=0.001  JointModeTransitionNonlinearIterations=2
  Solver Configuration : nesl_utility/Solver Configuration  PhysicalDomain=network_engine_domain  SubClassName=solver  LeftPortType=input  RightPortType=generic  Tones=[]  Harmonics=[]  SimulateNoise=off  Profile=off  UseLocalSampling=off  EnableSwitchedLinearOptims=on  FrequencyDomain=off  UseCCode=off  RelTol=0.001  AbsTol=1e-06  MinStep=1e-09  ToWorkspace=off  RevertToSquareIcSolve=off  NumHomotopyIterations=100  PhasorMode=off  PhasorModeNumHarmonics=1  ConsistencySolver=NEWTON_XTOL_AFTER_FTOL  CanonicalOrdering=UNORDERED  OptimizeIntermediates=UNOPTIMIZED  MulticoreSolverChoice=BACKWARD_EULER  IndexReductionMethod=DerivativeReplacement  DoDC=off  ResidualTolerance=1e-09  ConsistencyTolSource=GLOBAL  ConsistencyAbsTol=0.001  ConsistencyRelTol=0.001  ConsistencyTolFactor=0.001  UseLocalSolver=off  LocalSolverChoice=NE_BACKWARD_EULER_ADVANCER  ResolveIndetEquations=on  FunctionEvalNumThread=1  LocalSolverSampleTime=0.001  DoFixedCost=off  MaxNonlinIter=3  MaxModeIter=2  ComputeImpulses=off  ImpulseIterations=2  LinearAlgebra=Sparse  LinearAlgebraNumThread=0  EquationFormulation=NE_TIME_EF  DelaysMemoryBudget=1024  AutomaticFiltering=on  FilteringTimeConstant=0.001  PartitionStorageMethod=AS_NEEDED  PartitionMemoryBudget=1024  PartitionMethod=FAST  MultibodyUseLocalSolver=off  MultibodyLocalSolverChoice=ODE1  MultibodyLocalSolverSampleTime=0.001
  World Frame : sm_lib/Frames and Transforms/World Frame
  W : PMIOPort  Side=Left
  connections:
  Solver Configuration/RConn1 -- Mechanism Configuration/RConn1 -- W/RConn1 -- World Frame/RConn1

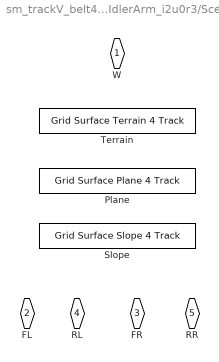
== system sm_trackV_belt4_IdlerArm_i2u0r3/Scene ==
  Plane : sm_trackV_lib_terrain_contact/Grid Surface Plane 4 Track  VariantControl=Plane  TranslationCartesianOffset=[1.5 17 0]  BrickDimensions=[28 40 0.05]
  Slope : sm_trackV_lib_terrain_contact/Grid Surface Slope 4 Track  VariantControl=Slope  road_len=Scene.Slope.road_len  road_wid=Scene.Slope.road_wid  slope_rise=Scene.Slope.slope_rise  slope_run=Scene.Slope.slope_run  slope_x0=Scene.Slope.slope_start  slope_xres=Scene.Slope.slope_xres  surface_clr=Scene.Slope.clr  surface_opc=Scene.Slope.opc  K_Road=Scene.Contact.Terrain.K  B_Road=Scene.Contact.Terrain.B  TW_Road=Scene.Contact.Terrain.TW  F_dyn_Road=Scene.Contact.Terrain.mud  F_stat_Road=Scene.Contact.Terrain.mus  CV_Road=Scene.Contact.Terrain.CV
  Terrain : sm_trackV_lib_terrain_contact/Grid Surface Terrain 4 Track  SystemSampleTime=-1  VariantControl=Terrain  VariantActivationTime=update diagram  EmptyChoice=off  PassThrough=off  PassThroughVariantControl=(default)  EmptyChoiceVariantControl=(default)  AllowFlexibleInterface=on  Latency=0  AutoFrameSizeCalculation=off
  W : PMIOPort  Side=Right
  FL : PMIOPort  Port=2  Side=Left
  FR : PMIOPort  Port=3  Side=Left
  RL : PMIOPort  Port=4  Side=Left
  RR : PMIOPort  Port=5  Side=Left

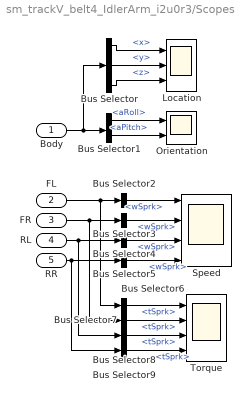
== system sm_trackV_belt4_IdlerArm_i2u0r3/Scopes ==
  Body : Inport
  FL : Inport  Port=2
  FR : Inport  Port=3
  RL : Inport  Port=4
  RR : Inport  Port=5
  Bus Selector : BusSelector  OutputSignals=x,y,z
  Bus Selector1 : BusSelector  OutputSignals=aRoll,aPitch
  Bus Selector{2..5} (4 alike) : BusSelector  OutputSignals=Underc.wSprk
  Bus Selector{6..9} (4 alike) : BusSelector  OutputSignals=Underc.tSprk
  Location : Scope  NumInputPorts=3
      settings: ActiveDisplayYMinimum=-2.438  ActiveDisplayYMaximum=13.72233
  Orientation : Scope  NumInputPorts=2
      settings: ActiveDisplayYMinimum=-0.40552  ActiveDisplayYMaximum=0.36121  DataLoggingVariableName=ScopeData2
  Speed : Scope  NumInputPorts=4
      settings: ActiveDisplayYMinimum=-0.59655  ActiveDisplayYMaximum=1.11207
  Torque : Scope  NumInputPorts=4
      settings: ActiveDisplayYMinimum=-13513.24622  ActiveDisplayYMaximum=6756.69226  DataLoggingVariableName=ScopeData2
  wires:
  Body/1 -> Bus Selector/1, Bus Selector1/1
  Bus Selector/3 -> Location/3  "<z>"
  RL/1 -> Bus Selector8/1, Bus Selector4/1
  Bus Selector1/1 -> Orientation/1  "<aRoll>"
  Bus Selector/2 -> Location/2  "<y>"
  Bus Selector/1 -> Location/1  "<x>"
  Bus Selector1/2 -> Orientation/2  "<aPitch>"
  RR/1 -> Bus Selector9/1, Bus Selector5/1
  FR/1 -> Bus Selector7/1, Bus Selector3/1
  FL/1 -> Bus Selector6/1, Bus Selector2/1
  Bus Selector2/1 -> Speed/1  "<wSprk>"
  Bus Selector3/1 -> Speed/2  "<wSprk>"
  Bus Selector4/1 -> Speed/3  "<wSprk>"
  Bus Selector5/1 -> Speed/4  "<wSprk>"
  Bus Selector6/1 -> Torque/1  "<tSprk>"
  Bus Selector7/1 -> Torque/2  "<tSprk>"
  Bus Selector8/1 -> Torque/3  "<tSprk>"
  Bus Selector9/1 -> Torque/4  "<tSprk>"

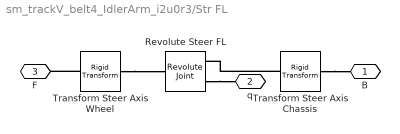
== system sm_trackV_belt4_IdlerArm_i2u0r3/Str FL ==
  Revolute Steer FL : sm_lib/Joints/Revolute Joint  JointMode=Normal  CompositeWrenchDir=FollowerOnBase  CompositeWrenchFrame=BaseFrame  SenseConstraintForce=off  SenseConstraintTorque=off  SenseTotalForce=off  SenseTotalTorque=off  PositionTargetSpecify=off  PositionTargetPriority=High  PositionTargetValue=0  PositionTargetValueUnits=deg  VelocityTargetSpecify=off  VelocityTargetPriority=High  VelocityTargetValue=0  VelocityTargetValueUnits=deg/s  EquilibriumPosition=0  EquilibriumPositionUnits=deg  SpringStiffness=0  SpringStiffnessUnits=N*m/deg  DampingCoefficient=0  DampingCoefficientUnits=N*m/(deg/s)  LowerLimitSpecify=off  LowerLimitBound=-90  LowerLimitBoundUnits=deg  LowerLimitStiffness=1e4  LowerLimitStiffnessUnits=N*m/deg  LowerLimitDamping=10  LowerLimitDampingUnits=N*m/(deg/s)  LowerLimitTransitionRegionWidth=0.1  LowerLimitTransitionRegionWidthUnits=deg  UpperLimitSpecify=off  UpperLimitBound=90  UpperLimitBoundUnits=deg  UpperLimitStiffness=1e4  UpperLimitStiffnessUnits=N*m/deg  UpperLimitDamping=10  UpperLimitDampingUnits=N*m/(deg/s)  UpperLimitTransitionRegionWidth=0.1  UpperLimitTransitionRegionWidthUnits=deg  TorqueActuationMode=ComputedTorque  MotionActuationMode=InputMotion  SensePosition=off  SenseVelocity=off  SenseAcceleration=off  SenseTorqueForce=off  SenseLowerLimitTorqueForce=off  SenseUpperLimitTorqueForce=off
  Transform Steer Axis Chassis : sm_lib/Frames and Transforms/Rigid Transform  RotationMethod=StandardAxis  FollAlignAxisA=+X  BaseAlignAxisA=+Y  FollAlignAxisB=+Y  BaseAlignAxisB=+Z  RotationStandardAxis=+X  RotationAngle=90  RotationAngleUnits=deg  RotationArbitraryAxis=[0 0 1]  RotationSequenceAxes=FollowerAxes  RotationSequence=XYX  RotationSequenceAngles=[0 0 0]  RotationSequenceAnglesUnits=deg  RotationMatrix=[1 0 0; 0 1 0; 0 0 1]  Quaternion=[1 0 0 0]  TranslationMethod=None  TranslationCartesianOffset=[0 0 0]  TranslationCartesianOffsetUnits=m  TranslationStandardAxis=+Z  TranslationStandardOffset=0  TranslationStandardOffsetUnits=m  TranslationROffset=0  TranslationROffsetUnits=m  TranslationThetaOffset=0  TranslationThetaOffsetUnits=deg  TranslationZOffset=0  TranslationZOffsetUnits=m
  Transform Steer Axis Wheel : sm_lib/Frames and Transforms/Rigid Transform  RotationMethod=StandardAxis  FollAlignAxisA=+X  BaseAlignAxisA=+Y  FollAlignAxisB=+Y  BaseAlignAxisB=+Z  RotationStandardAxis=+X  RotationAngle=90  RotationAngleUnits=deg  RotationArbitraryAxis=[0 0 1]  RotationSequenceAxes=FollowerAxes  RotationSequence=XYX  RotationSequenceAngles=[0 0 0]  RotationSequenceAnglesUnits=deg  RotationMatrix=[1 0 0; 0 1 0; 0 0 1]  Quaternion=[1 0 0 0]  TranslationMethod=None  TranslationCartesianOffset=[0 0 0]  TranslationCartesianOffsetUnits=m  TranslationStandardAxis=+Z  TranslationStandardOffset=0  TranslationStandardOffsetUnits=m  TranslationROffset=0  TranslationROffsetUnits=m  TranslationThetaOffset=0  TranslationThetaOffsetUnits=deg  TranslationZOffset=0  TranslationZOffsetUnits=m
  B : PMIOPort  Side=Left
  q : PMIOPort  Port=2  Side=Left
  F : PMIOPort  Port=3  Side=Right
  connections:
  Revolute Steer FL/LConn2 -- q/RConn1
  Transform Steer Axis Wheel/LConn1 -- F/RConn1
  Transform Steer Axis Chassis/LConn1 -- B/RConn1
  Transform Steer Axis Wheel/RConn1 -- Revolute Steer FL/RConn1
  Transform Steer Axis Chassis/RConn1 -- Revolute Steer FL/LConn1

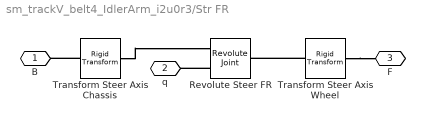
== system sm_trackV_belt4_IdlerArm_i2u0r3/Str FR ==
  Revolute Steer FR : sm_lib/Joints/Revolute Joint  JointMode=Normal  CompositeWrenchDir=FollowerOnBase  CompositeWrenchFrame=BaseFrame  SenseConstraintForce=off  SenseConstraintTorque=off  SenseTotalForce=off  SenseTotalTorque=off  PositionTargetSpecify=off  PositionTargetPriority=High  PositionTargetValue=0  PositionTargetValueUnits=deg  VelocityTargetSpecify=off  VelocityTargetPriority=High  VelocityTargetValue=0  VelocityTargetValueUnits=deg/s  EquilibriumPosition=0  EquilibriumPositionUnits=deg  SpringStiffness=0  SpringStiffnessUnits=N*m/deg  DampingCoefficient=0  DampingCoefficientUnits=N*m/(deg/s)  LowerLimitSpecify=off  LowerLimitBound=-90  LowerLimitBoundUnits=deg  LowerLimitStiffness=1e4  LowerLimitStiffnessUnits=N*m/deg  LowerLimitDamping=10  LowerLimitDampingUnits=N*m/(deg/s)  LowerLimitTransitionRegionWidth=0.1  LowerLimitTransitionRegionWidthUnits=deg  UpperLimitSpecify=off  UpperLimitBound=90  UpperLimitBoundUnits=deg  UpperLimitStiffness=1e4  UpperLimitStiffnessUnits=N*m/deg  UpperLimitDamping=10  UpperLimitDampingUnits=N*m/(deg/s)  UpperLimitTransitionRegionWidth=0.1  UpperLimitTransitionRegionWidthUnits=deg  TorqueActuationMode=ComputedTorque  MotionActuationMode=InputMotion  SensePosition=off  SenseVelocity=off  SenseAcceleration=off  SenseTorqueForce=off  SenseLowerLimitTorqueForce=off  SenseUpperLimitTorqueForce=off
  Transform Steer Axis Chassis : sm_lib/Frames and Transforms/Rigid Transform  RotationMethod=StandardAxis  FollAlignAxisA=+X  BaseAlignAxisA=+Y  FollAlignAxisB=+Y  BaseAlignAxisB=+Z  RotationStandardAxis=+X  RotationAngle=90  RotationAngleUnits=deg  RotationArbitraryAxis=[0 0 1]  RotationSequenceAxes=FollowerAxes  RotationSequence=XYX  RotationSequenceAngles=[0 0 0]  RotationSequenceAnglesUnits=deg  RotationMatrix=[1 0 0; 0 1 0; 0 0 1]  Quaternion=[1 0 0 0]  TranslationMethod=None  TranslationCartesianOffset=[0 0 0]  TranslationCartesianOffsetUnits=m  TranslationStandardAxis=+Z  TranslationStandardOffset=0  TranslationStandardOffsetUnits=m  TranslationROffset=0  TranslationROffsetUnits=m  TranslationThetaOffset=0  TranslationThetaOffsetUnits=deg  TranslationZOffset=0  TranslationZOffsetUnits=m
  Transform Steer Axis Wheel : sm_lib/Frames and Transforms/Rigid Transform  RotationMethod=StandardAxis  FollAlignAxisA=+X  BaseAlignAxisA=+Y  FollAlignAxisB=+Y  BaseAlignAxisB=+Z  RotationStandardAxis=+X  RotationAngle=90  RotationAngleUnits=deg  RotationArbitraryAxis=[0 0 1]  RotationSequenceAxes=FollowerAxes  RotationSequence=XYX  RotationSequenceAngles=[0 0 0]  RotationSequenceAnglesUnits=deg  RotationMatrix=[1 0 0; 0 1 0; 0 0 1]  Quaternion=[1 0 0 0]  TranslationMethod=None  TranslationCartesianOffset=[0 0 0]  TranslationCartesianOffsetUnits=m  TranslationStandardAxis=+Z  TranslationStandardOffset=0  TranslationStandardOffsetUnits=m  TranslationROffset=0  TranslationROffsetUnits=m  TranslationThetaOffset=0  TranslationThetaOffsetUnits=deg  TranslationZOffset=0  TranslationZOffsetUnits=m
  B : PMIOPort  Side=Left
  q : PMIOPort  Port=2  Side=Left
  F : PMIOPort  Port=3  Side=Right
  connections:
  Transform Steer Axis Chassis/RConn1 -- Revolute Steer FR/LConn1
  Transform Steer Axis Wheel/RConn1 -- Revolute Steer FR/RConn1
  Transform Steer Axis Chassis/LConn1 -- B/RConn1
  Transform Steer Axis Wheel/LConn1 -- F/RConn1
  Revolute Steer FR/LConn2 -- q/RConn1

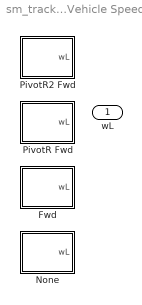
== system sm_trackV_belt4_IdlerArm_i2u0r3/Vehicle Speed ==
  Fwd : Subsystem  VariantControl=Fwd
  None : Subsystem  VariantControl=None
  PivotR Fwd : Subsystem  VariantControl=PivotR_Fwd
  PivotR2 Fwd : Subsystem  VariantControl=PivotR2_Fwd
  wL : Outport

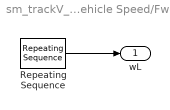
== system sm_trackV_belt4_IdlerArm_i2u0r3/Vehicle Speed/Fwd ==
  Repeating Sequence : simulink/Sources/Repeating Sequence  rep_seq_t=[0 2 2.01 60]  rep_seq_y=[0 0 3 3]
  wL : Outport
  wires:
  Repeating Sequence/1 -> wL/1

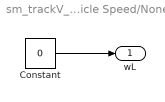
== system sm_trackV_belt4_IdlerArm_i2u0r3/Vehicle Speed/None ==
  Constant : Constant  Value=0
  wL : Outport
  wires:
  Constant/1 -> wL/1

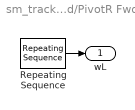
== system sm_trackV_belt4_IdlerArm_i2u0r3/Vehicle Speed/PivotR Fwd ==
  Repeating Sequence : simulink/Sources/Repeating Sequence  rep_seq_t=[0 2 2.01 40]  rep_seq_y=[0 0 3 3]
  wL : Outport
  wires:
  Repeating Sequence/1 -> wL/1

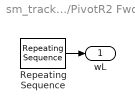
== system sm_trackV_belt4_IdlerArm_i2u0r3/Vehicle Speed/PivotR2 Fwd ==
  Repeating Sequence : simulink/Sources/Repeating Sequence  rep_seq_t=[0 2 2.01 40]  rep_seq_y=[0 0 3 3]
  wL : Outport
  wires:
  Repeating Sequence/1 -> wL/1
